simulink model "DPWMA_17_Level_Rectifier_Digital_PR"  (R2023b)
settings: Solver=VariableStepAuto  StartTime=0.0  StopTime=0.5  RelTol=1e-3
libraries: spsDiodeLib x144, spsSeriesRLCBranchLib x39, spsVoltageMeasurementLib x27, spsIGBTDiodeLib x24, simulink x12, spsACVoltageSourceLib x3, spsCurrentMeasurementLib x2, spsMeanLib x2, spsRMSLib x2, slpidlib x1, spsTHDLib x1, spspowerguiLib x1
(part 2 of 2)

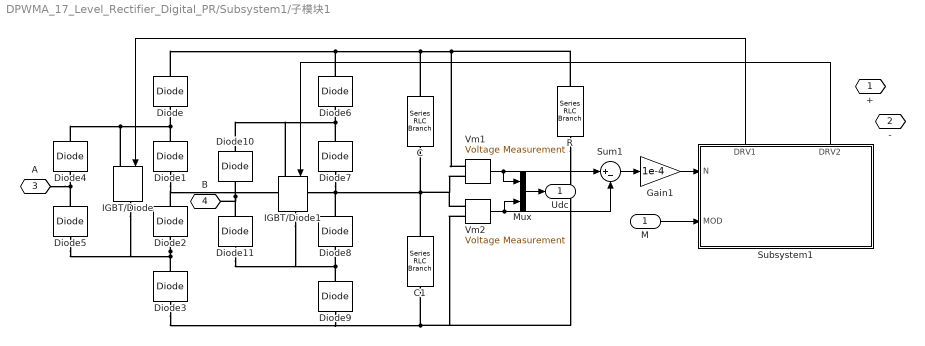
== system DPWMA_17_Level_Rectifier_Digital_PR/Subsystem1/子模块1 ==
  M : Inport
  C : spsSeriesRLCBranchLib/Series RLC Branch  LConnTagsString=__new0  RConnTagsString=__new0  BranchType=C  Resistance=0  Inductance=0  SetiL0=off  InitialCurrent=0  Capacitance=4e-3  Setx0=on  InitialVoltage=860  Measurements=None
  C1 : spsSeriesRLCBranchLib/Series RLC Branch  LConnTagsString=__new0  RConnTagsString=__new0  BranchType=C  Resistance=0  Inductance=0  SetiL0=off  InitialCurrent=0  Capacitance=4e-3  Setx0=on  InitialVoltage=860  Measurements=None
  Diode{,1..3,6..9} (8 alike) : spsDiodeLib/Diode  Ron=0.001  Lon=0  Vf=1.8  IC=0  UseSnubber=0  Rs=5e6  Cs=2e-9  Measurements=off
  Diode{4..5,10..11} (4 alike) : spsDiodeLib/Diode  Ron=0.001  Lon=0  Vf=1  IC=0  UseSnubber=0  Rs=0.05  Cs=1e-8  Measurements=off
  Gain1 : Gain  Gain=1e-4
  IGBT/Diode : spsIGBTDiodeLib/IGBT//Diode  Ron=1e-3  Rs=1e5  Cs=inf  Measurements=off
  IGBT/Diode1 : spsIGBTDiodeLib/IGBT//Diode  Ron=1e-3  Rs=1e5  Cs=inf  Measurements=off
  Mux : Mux  Inputs=2
  R : spsSeriesRLCBranchLib/Series RLC Branch  LConnTagsString=__new0  RConnTagsString=__new0  BranchType=R  Resistance=30  Inductance=0  SetiL0=off  InitialCurrent=0  Capacitance=2e-3  Setx0=on  InitialVoltage=311  Measurements=None
  Subsystem1 : Subsystem
      settings: PortSchema="{\"entries\":[{\"content\":{\"sides\":[{\"content\":{\"connectorIds\":[\"In1\",\"In2\"]},\"type\":\"ConnectorPlacement.EquallySpacedRectSide\",\"uuid\":\"86aef1ad-fbca-44c0-97c4-c9d179baa788\"},{\"content\":{\"side\":\"RIGHT\"},\"type\":\"ConnectorPlacement.EquallySpacedRectSide\",\"uuid\":\"7b15a0f8-39b1-4cc5-afe7-a687626936eb\"},{\"content\":{\"connectorIds\":[\"Out1\",\"Out2\"],\"side\":\"TOP\"},\"type\":\"ConnectorPlacement.EquallySpacedRectSide\",\"uuid\":\"a58ec6d0-3129-4061-af12-e971b5e0e948\"}]},\"type\":\"ConnectorPlacement.EquallySpacedConnector\",\"uuid\":\"d3f7daee-0424-497d-bc41-11931290c6fe\"}],\"packageUris\":[\"http://schema.mathworks.com/mf0/Connector/R2020b\"],\"version\":\"1.0\"}"
  Sum1 : Sum  Inputs=|+-
  Vm1 : spsVoltageMeasurementLib/Voltage Measurement  PhasorSimulation=off  OutputType=Complex  PSBequivalent=0
  Vm2 : spsVoltageMeasurementLib/Voltage Measurement  PhasorSimulation=off  OutputType=Complex  PSBequivalent=0
  + : PMIOPort  Side=Left
  - : PMIOPort  Port=2  Side=Left
  A : PMIOPort  Port=3  Side=Right
  B : PMIOPort  Port=4  Side=Right
  Udc : Outport
  wires:
  Subsystem1/2(DRV2) -> IGBT/Diode1/1
  Subsystem1/1(DRV1) -> IGBT/Diode/1
  M/1 -> Subsystem1/2(MOD)
  Mux/1 -> Udc/1
  Gain1/1 -> Subsystem1/1(N)
  Sum1/1 -> Gain1/1
  Vm2/1 -> Sum1/2, Mux/2
  Vm1/1 -> Sum1/1, Mux/1
  connections:
  Diode10/LConn1 -- B/RConn1 -- Diode11/RConn1
  Diode9/RConn1 -- Diode8/LConn1 -- IGBT/Diode1/RConn1 -- Diode11/LConn1
  Diode7/RConn1 -- Diode6/LConn1 -- Diode10/RConn1 -- IGBT/Diode1/LConn1
  A/RConn1 -- Diode5/RConn1 -- Diode4/LConn1
  Vm2/LConn2 -- R/RConn1 -- Diode3/LConn1 -- Diode9/LConn1 -- C1/RConn1
  Diode2/LConn1 -- Diode3/RConn1 -- Diode5/LConn1 -- IGBT/Diode/RConn1
  Diode4/RConn1 -- IGBT/Diode/LConn1 -- Diode1/RConn1 -- Diode/LConn1
  Diode7/LConn1 -- Diode2/RConn1 -- Diode1/LConn1 -- C/RConn1 -- C1/LConn1 -- Vm2/LConn1 -- Vm1/LConn2 -- Diode8/RConn1
  Diode6/RConn1 -- Diode/RConn1 -- C/LConn1 -- R/LConn1 -- Vm1/LConn1

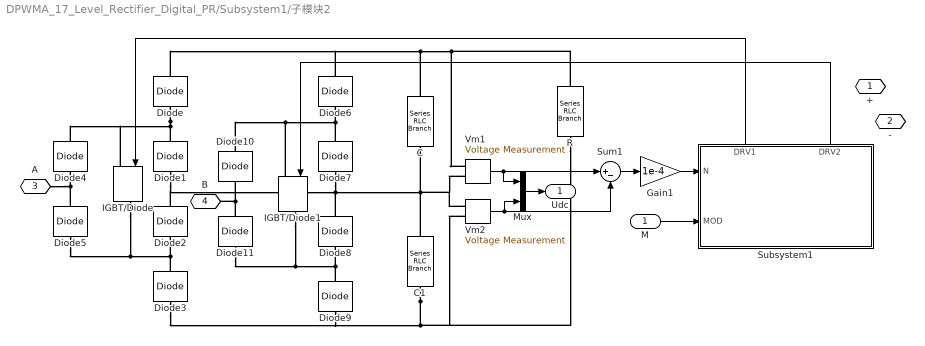
== system DPWMA_17_Level_Rectifier_Digital_PR/Subsystem1/子模块2 ==
  M : Inport
  C : spsSeriesRLCBranchLib/Series RLC Branch  LConnTagsString=__new0  RConnTagsString=__new0  BranchType=C  Resistance=0  Inductance=0  SetiL0=off  InitialCurrent=0  Capacitance=4e-3  Setx0=on  InitialVoltage=850  Measurements=None
  C1 : spsSeriesRLCBranchLib/Series RLC Branch  LConnTagsString=__new0  RConnTagsString=__new0  BranchType=C  Resistance=0  Inductance=0  SetiL0=off  InitialCurrent=0  Capacitance=4e-3  Setx0=on  InitialVoltage=850  Measurements=None
  Diode{,1..3,6..9} (8 alike) : spsDiodeLib/Diode  Ron=0.001  Lon=0  Vf=1.8  IC=0  UseSnubber=0  Rs=5e6  Cs=2e-9  Measurements=off
  Diode{4..5,10..11} (4 alike) : spsDiodeLib/Diode  Ron=0.001  Lon=0  Vf=1  IC=0  UseSnubber=0  Rs=0.05  Cs=1e-8  Measurements=off
  Gain1 : Gain  Gain=1e-4
  IGBT/Diode : spsIGBTDiodeLib/IGBT//Diode  Ron=1e-3  Rs=1e5  Cs=inf  Measurements=off
  IGBT/Diode1 : spsIGBTDiodeLib/IGBT//Diode  Ron=1e-3  Rs=1e5  Cs=inf  Measurements=off
  Mux : Mux  Inputs=2
  R : spsSeriesRLCBranchLib/Series RLC Branch  LConnTagsString=__new0  RConnTagsString=__new0  BranchType=R  Resistance=30  Inductance=0  SetiL0=off  InitialCurrent=0  Capacitance=2e-3  Setx0=on  InitialVoltage=311  Measurements=None
  Subsystem1 : Subsystem
      settings: PortSchema="{\"entries\":[{\"content\":{\"sides\":[{\"content\":{\"connectorIds\":[\"In1\",\"In2\"]},\"type\":\"ConnectorPlacement.EquallySpacedRectSide\",\"uuid\":\"86aef1ad-fbca-44c0-97c4-c9d179baa788\"},{\"content\":{\"side\":\"RIGHT\"},\"type\":\"ConnectorPlacement.EquallySpacedRectSide\",\"uuid\":\"7b15a0f8-39b1-4cc5-afe7-a687626936eb\"},{\"content\":{\"connectorIds\":[\"Out1\",\"Out2\"],\"side\":\"TOP\"},\"type\":\"ConnectorPlacement.EquallySpacedRectSide\",\"uuid\":\"a58ec6d0-3129-4061-af12-e971b5e0e948\"}]},\"type\":\"ConnectorPlacement.EquallySpacedConnector\",\"uuid\":\"d3f7daee-0424-497d-bc41-11931290c6fe\"}],\"packageUris\":[\"http://schema.mathworks.com/mf0/Connector/R2020b\"],\"version\":\"1.0\"}"
  Sum1 : Sum  Inputs=|+-
  Vm1 : spsVoltageMeasurementLib/Voltage Measurement  PhasorSimulation=off  OutputType=Complex  PSBequivalent=0
  Vm2 : spsVoltageMeasurementLib/Voltage Measurement  PhasorSimulation=off  OutputType=Complex  PSBequivalent=0
  + : PMIOPort  Side=Left
  - : PMIOPort  Port=2  Side=Left
  A : PMIOPort  Port=3  Side=Right
  B : PMIOPort  Port=4  Side=Right
  Udc : Outport
  wires:
  Vm1/1 -> Mux/1, Sum1/1
  Vm2/1 -> Mux/2, Sum1/2
  Sum1/1 -> Gain1/1
  Gain1/1 -> Subsystem1/1(N)
  Mux/1 -> Udc/1
  M/1 -> Subsystem1/2(MOD)
  Subsystem1/1(DRV1) -> IGBT/Diode/1
  Subsystem1/2(DRV2) -> IGBT/Diode1/1
  connections:
  Vm1/LConn1 -- R/LConn1 -- C/LConn1 -- Diode/RConn1 -- Diode6/RConn1
  Diode8/RConn1 -- Vm1/LConn2 -- Vm2/LConn1 -- C1/LConn1 -- C/RConn1 -- Diode1/LConn1 -- Diode2/RConn1 -- Diode7/LConn1
  Diode/LConn1 -- Diode1/RConn1 -- IGBT/Diode/LConn1 -- Diode4/RConn1
  IGBT/Diode/RConn1 -- Diode5/LConn1 -- Diode3/RConn1 -- Diode2/LConn1
  C1/RConn1 -- Diode9/LConn1 -- Diode3/LConn1 -- R/RConn1 -- Vm2/LConn2
  Diode4/LConn1 -- Diode5/RConn1 -- A/RConn1
  IGBT/Diode1/LConn1 -- Diode10/RConn1 -- Diode6/LConn1 -- Diode7/RConn1
  Diode11/LConn1 -- IGBT/Diode1/RConn1 -- Diode8/LConn1 -- Diode9/RConn1
  Diode11/RConn1 -- B/RConn1 -- Diode10/LConn1

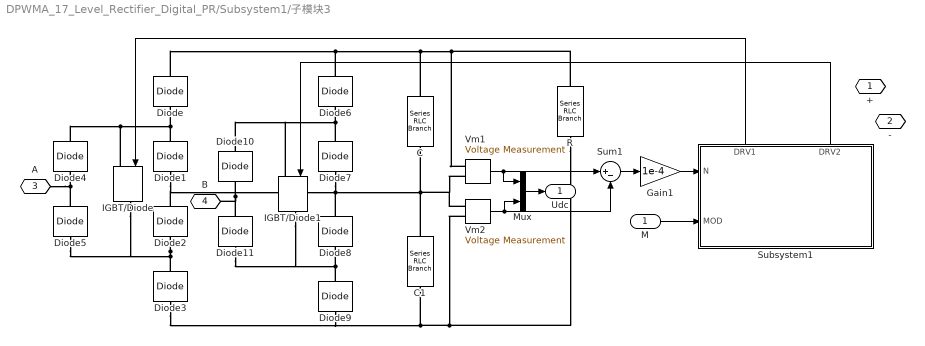
== system DPWMA_17_Level_Rectifier_Digital_PR/Subsystem1/子模块3 ==
  M : Inport
  C : spsSeriesRLCBranchLib/Series RLC Branch  LConnTagsString=__new0  RConnTagsString=__new0  BranchType=C  Resistance=0  Inductance=0  SetiL0=off  InitialCurrent=0  Capacitance=4e-3  Setx0=on  InitialVoltage=850  Measurements=None
  C1 : spsSeriesRLCBranchLib/Series RLC Branch  LConnTagsString=__new0  RConnTagsString=__new0  BranchType=C  Resistance=0  Inductance=0  SetiL0=off  InitialCurrent=0  Capacitance=4e-3  Setx0=on  InitialVoltage=850  Measurements=None
  Diode{,1..3,6..9} (8 alike) : spsDiodeLib/Diode  Ron=0.001  Lon=0  Vf=1.8  IC=0  UseSnubber=0  Rs=5e6  Cs=2e-9  Measurements=off
  Diode{4..5,10..11} (4 alike) : spsDiodeLib/Diode  Ron=0.001  Lon=0  Vf=1  IC=0  UseSnubber=0  Rs=0.05  Cs=1e-8  Measurements=off
  Gain1 : Gain  Gain=1e-4
  IGBT/Diode : spsIGBTDiodeLib/IGBT//Diode  Ron=1e-3  Rs=1e5  Cs=inf  Measurements=off
  IGBT/Diode1 : spsIGBTDiodeLib/IGBT//Diode  Ron=1e-3  Rs=1e5  Cs=inf  Measurements=off
  Mux : Mux  Inputs=2
  R : spsSeriesRLCBranchLib/Series RLC Branch  LConnTagsString=__new0  RConnTagsString=__new0  BranchType=R  Resistance=30  Inductance=0  SetiL0=off  InitialCurrent=0  Capacitance=2e-3  Setx0=on  InitialVoltage=311  Measurements=None
  Subsystem1 : Subsystem
      settings: PortSchema="{\"entries\":[{\"content\":{\"sides\":[{\"content\":{\"connectorIds\":[\"In1\",\"In2\"]},\"type\":\"ConnectorPlacement.EquallySpacedRectSide\",\"uuid\":\"86aef1ad-fbca-44c0-97c4-c9d179baa788\"},{\"content\":{\"side\":\"RIGHT\"},\"type\":\"ConnectorPlacement.EquallySpacedRectSide\",\"uuid\":\"7b15a0f8-39b1-4cc5-afe7-a687626936eb\"},{\"content\":{\"connectorIds\":[\"Out1\",\"Out2\"],\"side\":\"TOP\"},\"type\":\"ConnectorPlacement.EquallySpacedRectSide\",\"uuid\":\"a58ec6d0-3129-4061-af12-e971b5e0e948\"}]},\"type\":\"ConnectorPlacement.EquallySpacedConnector\",\"uuid\":\"d3f7daee-0424-497d-bc41-11931290c6fe\"}],\"packageUris\":[\"http://schema.mathworks.com/mf0/Connector/R2020b\"],\"version\":\"1.0\"}"
  Sum1 : Sum  Inputs=|+-
  Vm1 : spsVoltageMeasurementLib/Voltage Measurement  PhasorSimulation=off  OutputType=Complex  PSBequivalent=0
  Vm2 : spsVoltageMeasurementLib/Voltage Measurement  PhasorSimulation=off  OutputType=Complex  PSBequivalent=0
  + : PMIOPort  Side=Left
  - : PMIOPort  Port=2  Side=Left
  A : PMIOPort  Port=3  Side=Right
  B : PMIOPort  Port=4  Side=Right
  Udc : Outport
  wires:
  Subsystem1/2(DRV2) -> IGBT/Diode1/1
  Subsystem1/1(DRV1) -> IGBT/Diode/1
  M/1 -> Subsystem1/2(MOD)
  Mux/1 -> Udc/1
  Gain1/1 -> Subsystem1/1(N)
  Sum1/1 -> Gain1/1
  Vm2/1 -> Sum1/2, Mux/2
  Vm1/1 -> Sum1/1, Mux/1
  connections:
  Diode10/LConn1 -- B/RConn1 -- Diode11/RConn1
  Diode9/RConn1 -- Diode8/LConn1 -- IGBT/Diode1/RConn1 -- Diode11/LConn1
  Diode7/RConn1 -- Diode6/LConn1 -- Diode10/RConn1 -- IGBT/Diode1/LConn1
  A/RConn1 -- Diode5/RConn1 -- Diode4/LConn1
  Vm2/LConn2 -- R/RConn1 -- Diode3/LConn1 -- Diode9/LConn1 -- C1/RConn1
  Diode2/LConn1 -- Diode3/RConn1 -- Diode5/LConn1 -- IGBT/Diode/RConn1
  Diode4/RConn1 -- IGBT/Diode/LConn1 -- Diode1/RConn1 -- Diode/LConn1
  Diode7/LConn1 -- Diode2/RConn1 -- Diode1/LConn1 -- C/RConn1 -- C1/LConn1 -- Vm2/LConn1 -- Vm1/LConn2 -- Diode8/RConn1
  Diode6/RConn1 -- Diode/RConn1 -- C/LConn1 -- R/LConn1 -- Vm1/LConn1

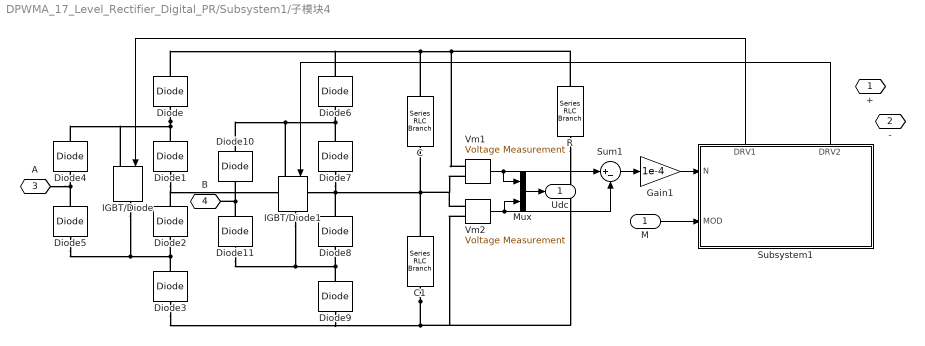
== system DPWMA_17_Level_Rectifier_Digital_PR/Subsystem1/子模块4 ==
  M : Inport
  C : spsSeriesRLCBranchLib/Series RLC Branch  LConnTagsString=__new0  RConnTagsString=__new0  BranchType=C  Resistance=0  Inductance=0  SetiL0=off  InitialCurrent=0  Capacitance=4e-3  Setx0=on  InitialVoltage=850  Measurements=None
  C1 : spsSeriesRLCBranchLib/Series RLC Branch  LConnTagsString=__new0  RConnTagsString=__new0  BranchType=C  Resistance=0  Inductance=0  SetiL0=off  InitialCurrent=0  Capacitance=4e-3  Setx0=on  InitialVoltage=850  Measurements=None
  Diode{,1..3,6..9} (8 alike) : spsDiodeLib/Diode  Ron=0.001  Lon=0  Vf=1.8  IC=0  UseSnubber=0  Rs=5e6  Cs=2e-9  Measurements=off
  Diode{4..5,10..11} (4 alike) : spsDiodeLib/Diode  Ron=0.001  Lon=0  Vf=1  IC=0  UseSnubber=0  Rs=0.05  Cs=1e-8  Measurements=off
  Gain1 : Gain  Gain=1e-4
  IGBT/Diode : spsIGBTDiodeLib/IGBT//Diode  Ron=1e-3  Rs=1e5  Cs=inf  Measurements=off
  IGBT/Diode1 : spsIGBTDiodeLib/IGBT//Diode  Ron=1e-3  Rs=1e5  Cs=inf  Measurements=off
  Mux : Mux  Inputs=2
  R : spsSeriesRLCBranchLib/Series RLC Branch  LConnTagsString=__new0  RConnTagsString=__new0  BranchType=R  Resistance=30  Inductance=0  SetiL0=off  InitialCurrent=0  Capacitance=2e-3  Setx0=on  InitialVoltage=311  Measurements=None
  Subsystem1 : Subsystem
      settings: PortSchema="{\"entries\":[{\"content\":{\"sides\":[{\"content\":{\"connectorIds\":[\"In1\",\"In2\"]},\"type\":\"ConnectorPlacement.EquallySpacedRectSide\",\"uuid\":\"86aef1ad-fbca-44c0-97c4-c9d179baa788\"},{\"content\":{\"side\":\"RIGHT\"},\"type\":\"ConnectorPlacement.EquallySpacedRectSide\",\"uuid\":\"7b15a0f8-39b1-4cc5-afe7-a687626936eb\"},{\"content\":{\"connectorIds\":[\"Out1\",\"Out2\"],\"side\":\"TOP\"},\"type\":\"ConnectorPlacement.EquallySpacedRectSide\",\"uuid\":\"a58ec6d0-3129-4061-af12-e971b5e0e948\"}]},\"type\":\"ConnectorPlacement.EquallySpacedConnector\",\"uuid\":\"d3f7daee-0424-497d-bc41-11931290c6fe\"}],\"packageUris\":[\"http://schema.mathworks.com/mf0/Connector/R2020b\"],\"version\":\"1.0\"}"
  Sum1 : Sum  Inputs=|+-
  Vm1 : spsVoltageMeasurementLib/Voltage Measurement  PhasorSimulation=off  OutputType=Complex  PSBequivalent=0
  Vm2 : spsVoltageMeasurementLib/Voltage Measurement  PhasorSimulation=off  OutputType=Complex  PSBequivalent=0
  + : PMIOPort  Side=Left
  - : PMIOPort  Port=2  Side=Left
  A : PMIOPort  Port=3  Side=Right
  B : PMIOPort  Port=4  Side=Right
  Udc : Outport
  wires:
  Vm1/1 -> Mux/1, Sum1/1
  Vm2/1 -> Mux/2, Sum1/2
  Sum1/1 -> Gain1/1
  Gain1/1 -> Subsystem1/1(N)
  Mux/1 -> Udc/1
  M/1 -> Subsystem1/2(MOD)
  Subsystem1/1(DRV1) -> IGBT/Diode/1
  Subsystem1/2(DRV2) -> IGBT/Diode1/1
  connections:
  Vm1/LConn1 -- R/LConn1 -- C/LConn1 -- Diode/RConn1 -- Diode6/RConn1
  Diode8/RConn1 -- Vm1/LConn2 -- Vm2/LConn1 -- C1/LConn1 -- C/RConn1 -- Diode1/LConn1 -- Diode2/RConn1 -- Diode7/LConn1
  Diode/LConn1 -- Diode1/RConn1 -- IGBT/Diode/LConn1 -- Diode4/RConn1
  IGBT/Diode/RConn1 -- Diode5/LConn1 -- Diode3/RConn1 -- Diode2/LConn1
  C1/RConn1 -- Diode9/LConn1 -- Diode3/LConn1 -- R/RConn1 -- Vm2/LConn2
  Diode4/LConn1 -- Diode5/RConn1 -- A/RConn1
  IGBT/Diode1/LConn1 -- Diode10/RConn1 -- Diode6/LConn1 -- Diode7/RConn1
  Diode11/LConn1 -- IGBT/Diode1/RConn1 -- Diode8/LConn1 -- Diode9/RConn1
  Diode11/RConn1 -- B/RConn1 -- Diode10/LConn1

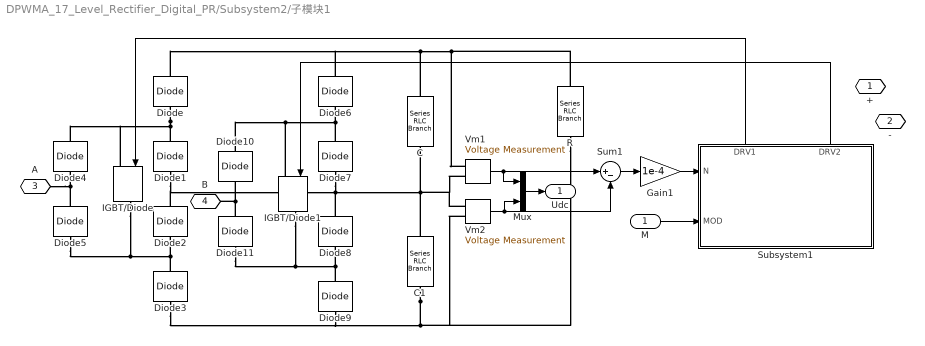
== system DPWMA_17_Level_Rectifier_Digital_PR/Subsystem2/子模块1 ==
  M : Inport
  C : spsSeriesRLCBranchLib/Series RLC Branch  LConnTagsString=__new0  RConnTagsString=__new0  BranchType=C  Resistance=0  Inductance=0  SetiL0=off  InitialCurrent=0  Capacitance=4e-3  Setx0=on  InitialVoltage=860  Measurements=None
  C1 : spsSeriesRLCBranchLib/Series RLC Branch  LConnTagsString=__new0  RConnTagsString=__new0  BranchType=C  Resistance=0  Inductance=0  SetiL0=off  InitialCurrent=0  Capacitance=4e-3  Setx0=on  InitialVoltage=860  Measurements=None
  Diode{,1..3,6..9} (8 alike) : spsDiodeLib/Diode  Ron=0.001  Lon=0  Vf=1.8  IC=0  UseSnubber=0  Rs=5e6  Cs=2e-9  Measurements=off
  Diode{4..5,10..11} (4 alike) : spsDiodeLib/Diode  Ron=0.001  Lon=0  Vf=1  IC=0  UseSnubber=0  Rs=0.05  Cs=1e-8  Measurements=off
  Gain1 : Gain  Gain=1e-4
  IGBT/Diode : spsIGBTDiodeLib/IGBT//Diode  Ron=1e-3  Rs=1e5  Cs=inf  Measurements=off
  IGBT/Diode1 : spsIGBTDiodeLib/IGBT//Diode  Ron=1e-3  Rs=1e5  Cs=inf  Measurements=off
  Mux : Mux  Inputs=2
  R : spsSeriesRLCBranchLib/Series RLC Branch  LConnTagsString=__new0  RConnTagsString=__new0  BranchType=R  Resistance=30  Inductance=0  SetiL0=off  InitialCurrent=0  Capacitance=2e-3  Setx0=on  InitialVoltage=311  Measurements=None
  Subsystem1 : Subsystem
      settings: PortSchema="{\"entries\":[{\"content\":{\"sides\":[{\"content\":{\"connectorIds\":[\"In1\",\"In2\"]},\"type\":\"ConnectorPlacement.EquallySpacedRectSide\",\"uuid\":\"86aef1ad-fbca-44c0-97c4-c9d179baa788\"},{\"content\":{\"side\":\"RIGHT\"},\"type\":\"ConnectorPlacement.EquallySpacedRectSide\",\"uuid\":\"7b15a0f8-39b1-4cc5-afe7-a687626936eb\"},{\"content\":{\"connectorIds\":[\"Out1\",\"Out2\"],\"side\":\"TOP\"},\"type\":\"ConnectorPlacement.EquallySpacedRectSide\",\"uuid\":\"a58ec6d0-3129-4061-af12-e971b5e0e948\"}]},\"type\":\"ConnectorPlacement.EquallySpacedConnector\",\"uuid\":\"d3f7daee-0424-497d-bc41-11931290c6fe\"}],\"packageUris\":[\"http://schema.mathworks.com/mf0/Connector/R2020b\"],\"version\":\"1.0\"}"
  Sum1 : Sum  Inputs=|+-
  Vm1 : spsVoltageMeasurementLib/Voltage Measurement  PhasorSimulation=off  OutputType=Complex  PSBequivalent=0
  Vm2 : spsVoltageMeasurementLib/Voltage Measurement  PhasorSimulation=off  OutputType=Complex  PSBequivalent=0
  + : PMIOPort  Side=Left
  - : PMIOPort  Port=2  Side=Left
  A : PMIOPort  Port=3  Side=Right
  B : PMIOPort  Port=4  Side=Right
  Udc : Outport
  wires:
  Vm1/1 -> Mux/1, Sum1/1
  Vm2/1 -> Mux/2, Sum1/2
  Sum1/1 -> Gain1/1
  Gain1/1 -> Subsystem1/1(N)
  Mux/1 -> Udc/1
  M/1 -> Subsystem1/2(MOD)
  Subsystem1/1(DRV1) -> IGBT/Diode/1
  Subsystem1/2(DRV2) -> IGBT/Diode1/1
  connections:
  Vm1/LConn1 -- R/LConn1 -- C/LConn1 -- Diode/RConn1 -- Diode6/RConn1
  Diode8/RConn1 -- Vm1/LConn2 -- Vm2/LConn1 -- C1/LConn1 -- C/RConn1 -- Diode1/LConn1 -- Diode2/RConn1 -- Diode7/LConn1
  Diode/LConn1 -- Diode1/RConn1 -- IGBT/Diode/LConn1 -- Diode4/RConn1
  IGBT/Diode/RConn1 -- Diode5/LConn1 -- Diode3/RConn1 -- Diode2/LConn1
  C1/RConn1 -- Diode9/LConn1 -- Diode3/LConn1 -- R/RConn1 -- Vm2/LConn2
  Diode4/LConn1 -- Diode5/RConn1 -- A/RConn1
  IGBT/Diode1/LConn1 -- Diode10/RConn1 -- Diode6/LConn1 -- Diode7/RConn1
  Diode11/LConn1 -- IGBT/Diode1/RConn1 -- Diode8/LConn1 -- Diode9/RConn1
  Diode11/RConn1 -- B/RConn1 -- Diode10/LConn1

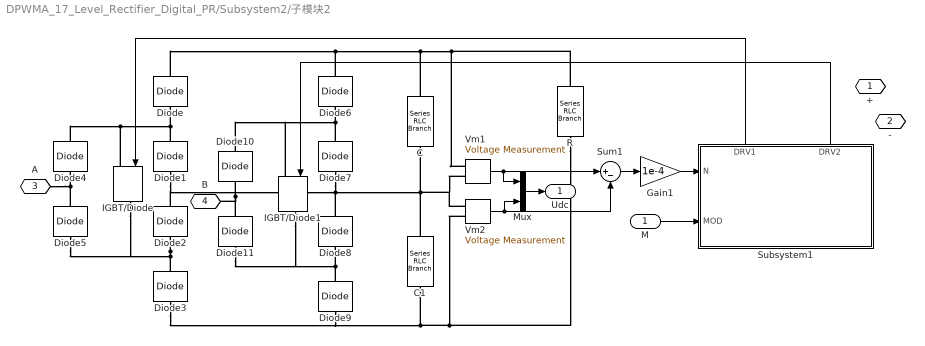
== system DPWMA_17_Level_Rectifier_Digital_PR/Subsystem2/子模块2 ==
  M : Inport
  C : spsSeriesRLCBranchLib/Series RLC Branch  LConnTagsString=__new0  RConnTagsString=__new0  BranchType=C  Resistance=0  Inductance=0  SetiL0=off  InitialCurrent=0  Capacitance=4e-3  Setx0=on  InitialVoltage=850  Measurements=None
  C1 : spsSeriesRLCBranchLib/Series RLC Branch  LConnTagsString=__new0  RConnTagsString=__new0  BranchType=C  Resistance=0  Inductance=0  SetiL0=off  InitialCurrent=0  Capacitance=4e-3  Setx0=on  InitialVoltage=850  Measurements=None
  Diode{,1..3,6..9} (8 alike) : spsDiodeLib/Diode  Ron=0.001  Lon=0  Vf=1.8  IC=0  UseSnubber=0  Rs=5e6  Cs=2e-9  Measurements=off
  Diode{4..5,10..11} (4 alike) : spsDiodeLib/Diode  Ron=0.001  Lon=0  Vf=1  IC=0  UseSnubber=0  Rs=0.05  Cs=1e-8  Measurements=off
  Gain1 : Gain  Gain=1e-4
  IGBT/Diode : spsIGBTDiodeLib/IGBT//Diode  Ron=1e-3  Rs=1e5  Cs=inf  Measurements=off
  IGBT/Diode1 : spsIGBTDiodeLib/IGBT//Diode  Ron=1e-3  Rs=1e5  Cs=inf  Measurements=off
  Mux : Mux  Inputs=2
  R : spsSeriesRLCBranchLib/Series RLC Branch  LConnTagsString=__new0  RConnTagsString=__new0  BranchType=R  Resistance=30  Inductance=0  SetiL0=off  InitialCurrent=0  Capacitance=2e-3  Setx0=on  InitialVoltage=311  Measurements=None
  Subsystem1 : Subsystem
      settings: PortSchema="{\"entries\":[{\"content\":{\"sides\":[{\"content\":{\"connectorIds\":[\"In1\",\"In2\"]},\"type\":\"ConnectorPlacement.EquallySpacedRectSide\",\"uuid\":\"86aef1ad-fbca-44c0-97c4-c9d179baa788\"},{\"content\":{\"side\":\"RIGHT\"},\"type\":\"ConnectorPlacement.EquallySpacedRectSide\",\"uuid\":\"7b15a0f8-39b1-4cc5-afe7-a687626936eb\"},{\"content\":{\"connectorIds\":[\"Out1\",\"Out2\"],\"side\":\"TOP\"},\"type\":\"ConnectorPlacement.EquallySpacedRectSide\",\"uuid\":\"a58ec6d0-3129-4061-af12-e971b5e0e948\"}]},\"type\":\"ConnectorPlacement.EquallySpacedConnector\",\"uuid\":\"d3f7daee-0424-497d-bc41-11931290c6fe\"}],\"packageUris\":[\"http://schema.mathworks.com/mf0/Connector/R2020b\"],\"version\":\"1.0\"}"
  Sum1 : Sum  Inputs=|+-
  Vm1 : spsVoltageMeasurementLib/Voltage Measurement  PhasorSimulation=off  OutputType=Complex  PSBequivalent=0
  Vm2 : spsVoltageMeasurementLib/Voltage Measurement  PhasorSimulation=off  OutputType=Complex  PSBequivalent=0
  + : PMIOPort  Side=Left
  - : PMIOPort  Port=2  Side=Left
  A : PMIOPort  Port=3  Side=Right
  B : PMIOPort  Port=4  Side=Right
  Udc : Outport
  wires:
  Subsystem1/2(DRV2) -> IGBT/Diode1/1
  Subsystem1/1(DRV1) -> IGBT/Diode/1
  M/1 -> Subsystem1/2(MOD)
  Mux/1 -> Udc/1
  Gain1/1 -> Subsystem1/1(N)
  Sum1/1 -> Gain1/1
  Vm2/1 -> Sum1/2, Mux/2
  Vm1/1 -> Sum1/1, Mux/1
  connections:
  Diode10/LConn1 -- B/RConn1 -- Diode11/RConn1
  Diode9/RConn1 -- Diode8/LConn1 -- IGBT/Diode1/RConn1 -- Diode11/LConn1
  Diode7/RConn1 -- Diode6/LConn1 -- Diode10/RConn1 -- IGBT/Diode1/LConn1
  A/RConn1 -- Diode5/RConn1 -- Diode4/LConn1
  Vm2/LConn2 -- R/RConn1 -- Diode3/LConn1 -- Diode9/LConn1 -- C1/RConn1
  Diode2/LConn1 -- Diode3/RConn1 -- Diode5/LConn1 -- IGBT/Diode/RConn1
  Diode4/RConn1 -- IGBT/Diode/LConn1 -- Diode1/RConn1 -- Diode/LConn1
  Diode7/LConn1 -- Diode2/RConn1 -- Diode1/LConn1 -- C/RConn1 -- C1/LConn1 -- Vm2/LConn1 -- Vm1/LConn2 -- Diode8/RConn1
  Diode6/RConn1 -- Diode/RConn1 -- C/LConn1 -- R/LConn1 -- Vm1/LConn1

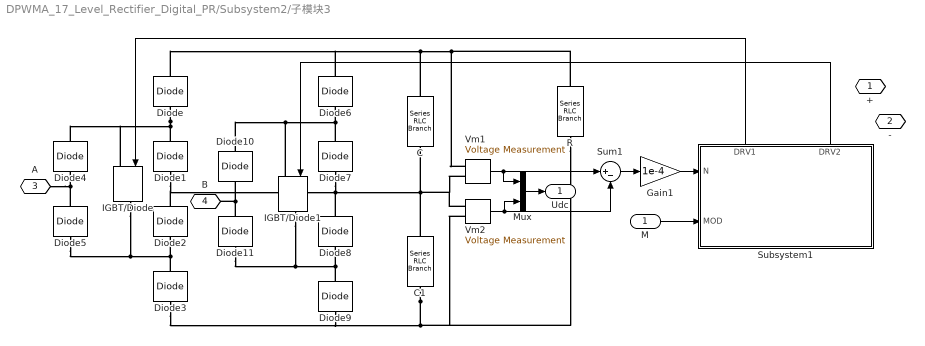
== system DPWMA_17_Level_Rectifier_Digital_PR/Subsystem2/子模块3 ==
  M : Inport
  C : spsSeriesRLCBranchLib/Series RLC Branch  LConnTagsString=__new0  RConnTagsString=__new0  BranchType=C  Resistance=0  Inductance=0  SetiL0=off  InitialCurrent=0  Capacitance=4e-3  Setx0=on  InitialVoltage=850  Measurements=None
  C1 : spsSeriesRLCBranchLib/Series RLC Branch  LConnTagsString=__new0  RConnTagsString=__new0  BranchType=C  Resistance=0  Inductance=0  SetiL0=off  InitialCurrent=0  Capacitance=4e-3  Setx0=on  InitialVoltage=850  Measurements=None
  Diode{,1..3,6..9} (8 alike) : spsDiodeLib/Diode  Ron=0.001  Lon=0  Vf=1.8  IC=0  UseSnubber=0  Rs=5e6  Cs=2e-9  Measurements=off
  Diode{4..5,10..11} (4 alike) : spsDiodeLib/Diode  Ron=0.001  Lon=0  Vf=1  IC=0  UseSnubber=0  Rs=0.05  Cs=1e-8  Measurements=off
  Gain1 : Gain  Gain=1e-4
  IGBT/Diode : spsIGBTDiodeLib/IGBT//Diode  Ron=1e-3  Rs=1e5  Cs=inf  Measurements=off
  IGBT/Diode1 : spsIGBTDiodeLib/IGBT//Diode  Ron=1e-3  Rs=1e5  Cs=inf  Measurements=off
  Mux : Mux  Inputs=2
  R : spsSeriesRLCBranchLib/Series RLC Branch  LConnTagsString=__new0  RConnTagsString=__new0  BranchType=R  Resistance=30  Inductance=0  SetiL0=off  InitialCurrent=0  Capacitance=2e-3  Setx0=on  InitialVoltage=311  Measurements=None
  Subsystem1 : Subsystem
      settings: PortSchema="{\"entries\":[{\"content\":{\"sides\":[{\"content\":{\"connectorIds\":[\"In1\",\"In2\"]},\"type\":\"ConnectorPlacement.EquallySpacedRectSide\",\"uuid\":\"86aef1ad-fbca-44c0-97c4-c9d179baa788\"},{\"content\":{\"side\":\"RIGHT\"},\"type\":\"ConnectorPlacement.EquallySpacedRectSide\",\"uuid\":\"7b15a0f8-39b1-4cc5-afe7-a687626936eb\"},{\"content\":{\"connectorIds\":[\"Out1\",\"Out2\"],\"side\":\"TOP\"},\"type\":\"ConnectorPlacement.EquallySpacedRectSide\",\"uuid\":\"a58ec6d0-3129-4061-af12-e971b5e0e948\"}]},\"type\":\"ConnectorPlacement.EquallySpacedConnector\",\"uuid\":\"d3f7daee-0424-497d-bc41-11931290c6fe\"}],\"packageUris\":[\"http://schema.mathworks.com/mf0/Connector/R2020b\"],\"version\":\"1.0\"}"
  Sum1 : Sum  Inputs=|+-
  Vm1 : spsVoltageMeasurementLib/Voltage Measurement  PhasorSimulation=off  OutputType=Complex  PSBequivalent=0
  Vm2 : spsVoltageMeasurementLib/Voltage Measurement  PhasorSimulation=off  OutputType=Complex  PSBequivalent=0
  + : PMIOPort  Side=Left
  - : PMIOPort  Port=2  Side=Left
  A : PMIOPort  Port=3  Side=Right
  B : PMIOPort  Port=4  Side=Right
  Udc : Outport
  wires:
  Vm1/1 -> Mux/1, Sum1/1
  Vm2/1 -> Mux/2, Sum1/2
  Sum1/1 -> Gain1/1
  Gain1/1 -> Subsystem1/1(N)
  Mux/1 -> Udc/1
  M/1 -> Subsystem1/2(MOD)
  Subsystem1/1(DRV1) -> IGBT/Diode/1
  Subsystem1/2(DRV2) -> IGBT/Diode1/1
  connections:
  Vm1/LConn1 -- R/LConn1 -- C/LConn1 -- Diode/RConn1 -- Diode6/RConn1
  Diode8/RConn1 -- Vm1/LConn2 -- Vm2/LConn1 -- C1/LConn1 -- C/RConn1 -- Diode1/LConn1 -- Diode2/RConn1 -- Diode7/LConn1
  Diode/LConn1 -- Diode1/RConn1 -- IGBT/Diode/LConn1 -- Diode4/RConn1
  IGBT/Diode/RConn1 -- Diode5/LConn1 -- Diode3/RConn1 -- Diode2/LConn1
  C1/RConn1 -- Diode9/LConn1 -- Diode3/LConn1 -- R/RConn1 -- Vm2/LConn2
  Diode4/LConn1 -- Diode5/RConn1 -- A/RConn1
  IGBT/Diode1/LConn1 -- Diode10/RConn1 -- Diode6/LConn1 -- Diode7/RConn1
  Diode11/LConn1 -- IGBT/Diode1/RConn1 -- Diode8/LConn1 -- Diode9/RConn1
  Diode11/RConn1 -- B/RConn1 -- Diode10/LConn1

== system DPWMA_17_Level_Rectifier_Digital_PR/Subsystem2/子模块4 ==
  M : Inport
  C : spsSeriesRLCBranchLib/Series RLC Branch  LConnTagsString=__new0  RConnTagsString=__new0  BranchType=C  Resistance=0  Inductance=0  SetiL0=off  InitialCurrent=0  Capacitance=4e-3  Setx0=on  InitialVoltage=850  Measurements=None
  C1 : spsSeriesRLCBranchLib/Series RLC Branch  LConnTagsString=__new0  RConnTagsString=__new0  BranchType=C  Resistance=0  Inductance=0  SetiL0=off  InitialCurrent=0  Capacitance=4e-3  Setx0=on  InitialVoltage=850  Measurements=None
  Diode{,1..3,6..9} (8 alike) : spsDiodeLib/Diode  Ron=0.001  Lon=0  Vf=1.8  IC=0  UseSnubber=0  Rs=5e6  Cs=2e-9  Measurements=off
  Diode{4..5,10..11} (4 alike) : spsDiodeLib/Diode  Ron=0.001  Lon=0  Vf=1  IC=0  UseSnubber=0  Rs=0.05  Cs=1e-8  Measurements=off
  Gain1 : Gain  Gain=1e-4
  IGBT/Diode : spsIGBTDiodeLib/IGBT//Diode  Ron=1e-3  Rs=1e5  Cs=inf  Measurements=off
  IGBT/Diode1 : spsIGBTDiodeLib/IGBT//Diode  Ron=1e-3  Rs=1e5  Cs=inf  Measurements=off
  Mux : Mux  Inputs=2
  R : spsSeriesRLCBranchLib/Series RLC Branch  LConnTagsString=__new0  RConnTagsString=__new0  BranchType=R  Resistance=30  Inductance=0  SetiL0=off  InitialCurrent=0  Capacitance=2e-3  Setx0=on  InitialVoltage=311  Measurements=None
  Subsystem1 : Subsystem
      settings: PortSchema="{\"entries\":[{\"content\":{\"sides\":[{\"content\":{\"connectorIds\":[\"In1\",\"In2\"]},\"type\":\"ConnectorPlacement.EquallySpacedRectSide\",\"uuid\":\"86aef1ad-fbca-44c0-97c4-c9d179baa788\"},{\"content\":{\"side\":\"RIGHT\"},\"type\":\"ConnectorPlacement.EquallySpacedRectSide\",\"uuid\":\"7b15a0f8-39b1-4cc5-afe7-a687626936eb\"},{\"content\":{\"connectorIds\":[\"Out1\",\"Out2\"],\"side\":\"TOP\"},\"type\":\"ConnectorPlacement.EquallySpacedRectSide\",\"uuid\":\"a58ec6d0-3129-4061-af12-e971b5e0e948\"}]},\"type\":\"ConnectorPlacement.EquallySpacedConnector\",\"uuid\":\"d3f7daee-0424-497d-bc41-11931290c6fe\"}],\"packageUris\":[\"http://schema.mathworks.com/mf0/Connector/R2020b\"],\"version\":\"1.0\"}"
  Sum1 : Sum  Inputs=|+-
  Vm1 : spsVoltageMeasurementLib/Voltage Measurement  PhasorSimulation=off  OutputType=Complex  PSBequivalent=0
  Vm2 : spsVoltageMeasurementLib/Voltage Measurement  PhasorSimulation=off  OutputType=Complex  PSBequivalent=0
  + : PMIOPort  Side=Left
  - : PMIOPort  Port=2  Side=Left
  A : PMIOPort  Port=3  Side=Right
  B : PMIOPort  Port=4  Side=Right
  Udc : Outport
  wires:
  Subsystem1/2(DRV2) -> IGBT/Diode1/1
  Subsystem1/1(DRV1) -> IGBT/Diode/1
  M/1 -> Subsystem1/2(MOD)
  Mux/1 -> Udc/1
  Gain1/1 -> Subsystem1/1(N)
  Sum1/1 -> Gain1/1
  Vm2/1 -> Sum1/2, Mux/2
  Vm1/1 -> Sum1/1, Mux/1
  connections:
  Diode10/LConn1 -- B/RConn1 -- Diode11/RConn1
  Diode9/RConn1 -- Diode8/LConn1 -- IGBT/Diode1/RConn1 -- Diode11/LConn1
  Diode7/RConn1 -- Diode6/LConn1 -- Diode10/RConn1 -- IGBT/Diode1/LConn1
  A/RConn1 -- Diode5/RConn1 -- Diode4/LConn1
  Vm2/LConn2 -- R/RConn1 -- Diode3/LConn1 -- Diode9/LConn1 -- C1/RConn1
  Diode2/LConn1 -- Diode3/RConn1 -- Diode5/LConn1 -- IGBT/Diode/RConn1
  Diode4/RConn1 -- IGBT/Diode/LConn1 -- Diode1/RConn1 -- Diode/LConn1
  Diode7/LConn1 -- Diode2/RConn1 -- Diode1/LConn1 -- C/RConn1 -- C1/LConn1 -- Vm2/LConn1 -- Vm1/LConn2 -- Diode8/RConn1
  Diode6/RConn1 -- Diode/RConn1 -- C/LConn1 -- R/LConn1 -- Vm1/LConn1

== system DPWMA_17_Level_Rectifier_Digital_PR/Subsystem3/QuTrans ==
  ac : Inport
  Demux : Demux  Outputs=2
  Mux : Mux  Inputs=3
  Sum6 : Sum  Inputs=-|-
  abc : Outport
  wires:
  ac/1 -> Demux/1
  Sum6/1 -> Mux/2
  Demux/1 -> Sum6/1, Mux/1
  Demux/2 -> Sum6/2, Mux/3
  Mux/1 -> abc/1

== system DPWMA_17_Level_Rectifier_Digital_PR/Subsystem3/QuTrans1 ==
  ac : Inport
  Demux : Demux  Outputs=2
  Mux : Mux  Inputs=3
  Sum6 : Sum  Inputs=-|-
  abc : Outport
  wires:
  Mux/1 -> abc/1
  Demux/2 -> Mux/3, Sum6/2
  Demux/1 -> Mux/1, Sum6/1
  Sum6/1 -> Mux/2
  ac/1 -> Demux/1

== system DPWMA_17_Level_Rectifier_Digital_PR/Subsystem/子模块1/Subsystem1 ==
  N : Inport
  MOD : Inport  Port=2
  AND : Logic  IconShape=distinctive  AllPortsSameDT=off  OutDataTypeStr=boolean
  AND1 : Logic  IconShape=distinctive  AllPortsSameDT=off  OutDataTypeStr=boolean
  OFFSET : Constant
  Relational Operator1 : RelationalOperator  Operator=<  OutDataTypeStr=boolean  InputSameDT=off
  Relational Operator2 : RelationalOperator  Operator=>  OutDataTypeStr=boolean  InputSameDT=off
  Relational Operator6 : RelationalOperator  Operator=>  OutDataTypeStr=boolean  InputSameDT=off
  Relational Operator7 : RelationalOperator  Operator=<  OutDataTypeStr=boolean  InputSameDT=off
  Sum1 : Sum  Inputs=|+-
  Sum2 : Sum  Inputs=|++
  Sum3 : Sum  Inputs=--|
  Sum4 : Sum  Inputs=++|
  Triangle1 : simulink/Sources/Repeating Sequence  rep_seq_t=[0 1/1800/2 1/1800]  rep_seq_y=[0 1 0]
  DRV1 : Outport
  DRV2 : Outport  Port=2
  wires:
  N/1 -> Sum3/1, Sum1/2
  MOD/1 -> Sum3/2, Sum1/1
  Sum1/1 -> Relational Operator7/1, Sum2/1
  Triangle1/1 -> Relational Operator2/2, Relational Operator1/2, Relational Operator6/2, Relational Operator7/2
  Sum2/1 -> Relational Operator6/1
  OFFSET/1 -> Sum2/2, Sum4/1
  Sum4/1 -> Relational Operator2/1
  Sum3/1 -> Relational Operator1/1, Sum4/2
  Relational Operator6/1 -> AND/2
  Relational Operator7/1 -> AND/1
  AND/1 -> DRV1/1
  Relational Operator1/1 -> AND1/1
  Relational Operator2/1 -> AND1/2
  AND1/1 -> DRV2/1

== system DPWMA_17_Level_Rectifier_Digital_PR/Subsystem/子模块2/Subsystem1 ==
  N : Inport
  MOD : Inport  Port=2
  AND : Logic  IconShape=distinctive  AllPortsSameDT=off  OutDataTypeStr=boolean
  AND1 : Logic  IconShape=distinctive  AllPortsSameDT=off  OutDataTypeStr=boolean
  OFFSET : Constant
  Relational Operator1 : RelationalOperator  Operator=<  OutDataTypeStr=boolean  InputSameDT=off
  Relational Operator2 : RelationalOperator  Operator=>  OutDataTypeStr=boolean  InputSameDT=off
  Relational Operator6 : RelationalOperator  Operator=>  OutDataTypeStr=boolean  InputSameDT=off
  Relational Operator7 : RelationalOperator  Operator=<  OutDataTypeStr=boolean  InputSameDT=off
  Sum1 : Sum  Inputs=|+-
  Sum2 : Sum  Inputs=|++
  Sum3 : Sum  Inputs=--|
  Sum4 : Sum  Inputs=++|
  Transport Delay : TransportDelay  DelayTime=1/3600/4
  Triangle1 : simulink/Sources/Repeating Sequence  rep_seq_t=[0 1/1800/2 1/1800]  rep_seq_y=[0 1 0]
  DRV1 : Outport
  DRV2 : Outport  Port=2
  wires:
  AND1/1 -> DRV2/1
  Relational Operator2/1 -> AND1/2
  Relational Operator1/1 -> AND1/1
  AND/1 -> DRV1/1
  Relational Operator7/1 -> AND/1
  Relational Operator6/1 -> AND/2
  Sum3/1 -> Sum4/2, Relational Operator1/1
  Sum4/1 -> Relational Operator2/1
  OFFSET/1 -> Sum4/1, Sum2/2
  Sum2/1 -> Relational Operator6/1
  Transport Delay/1 -> Relational Operator7/2, Relational Operator6/2, Relational Operator1/2, Relational Operator2/2
  Sum1/1 -> Sum2/1, Relational Operator7/1
  MOD/1 -> Sum1/1, Sum3/2
  N/1 -> Sum1/2, Sum3/1
  Triangle1/1 -> Transport Delay/1

== system DPWMA_17_Level_Rectifier_Digital_PR/Subsystem/子模块3/Subsystem1 ==
  N : Inport
  MOD : Inport  Port=2
  AND : Logic  IconShape=distinctive  AllPortsSameDT=off  OutDataTypeStr=boolean
  AND1 : Logic  IconShape=distinctive  AllPortsSameDT=off  OutDataTypeStr=boolean
  OFFSET : Constant
  Relational Operator1 : RelationalOperator  Operator=<  OutDataTypeStr=boolean  InputSameDT=off
  Relational Operator2 : RelationalOperator  Operator=>  OutDataTypeStr=boolean  InputSameDT=off
  Relational Operator6 : RelationalOperator  Operator=>  OutDataTypeStr=boolean  InputSameDT=off
  Relational Operator7 : RelationalOperator  Operator=<  OutDataTypeStr=boolean  InputSameDT=off
  Sum1 : Sum  Inputs=|+-
  Sum2 : Sum  Inputs=|++
  Sum3 : Sum  Inputs=--|
  Sum4 : Sum  Inputs=++|
  Transport Delay : TransportDelay  DelayTime=2/3600/4
  Triangle1 : simulink/Sources/Repeating Sequence  rep_seq_t=[0 1/1800/2 1/1800]  rep_seq_y=[0 1 0]
  DRV1 : Outport
  DRV2 : Outport  Port=2
  wires:
  Triangle1/1 -> Transport Delay/1
  N/1 -> Sum3/1, Sum1/2
  MOD/1 -> Sum3/2, Sum1/1
  Sum1/1 -> Relational Operator7/1, Sum2/1
  Transport Delay/1 -> Relational Operator2/2, Relational Operator1/2, Relational Operator6/2, Relational Operator7/2
  Sum2/1 -> Relational Operator6/1
  OFFSET/1 -> Sum2/2, Sum4/1
  Sum4/1 -> Relational Operator2/1
  Sum3/1 -> Relational Operator1/1, Sum4/2
  Relational Operator6/1 -> AND/2
  Relational Operator7/1 -> AND/1
  AND/1 -> DRV1/1
  Relational Operator1/1 -> AND1/1
  Relational Operator2/1 -> AND1/2
  AND1/1 -> DRV2/1

== system DPWMA_17_Level_Rectifier_Digital_PR/Subsystem/子模块4/Subsystem1 ==
  N : Inport
  MOD : Inport  Port=2
  AND : Logic  IconShape=distinctive  AllPortsSameDT=off  OutDataTypeStr=boolean
  AND1 : Logic  IconShape=distinctive  AllPortsSameDT=off  OutDataTypeStr=boolean
  OFFSET : Constant
  Relational Operator1 : RelationalOperator  Operator=<  OutDataTypeStr=boolean  InputSameDT=off
  Relational Operator2 : RelationalOperator  Operator=>  OutDataTypeStr=boolean  InputSameDT=off
  Relational Operator6 : RelationalOperator  Operator=>  OutDataTypeStr=boolean  InputSameDT=off
  Relational Operator7 : RelationalOperator  Operator=<  OutDataTypeStr=boolean  InputSameDT=off
  Sum1 : Sum  Inputs=|+-
  Sum2 : Sum  Inputs=|++
  Sum3 : Sum  Inputs=--|
  Sum4 : Sum  Inputs=++|
  Transport Delay : TransportDelay  DelayTime=3/3600/4
  Triangle1 : simulink/Sources/Repeating Sequence  rep_seq_t=[0 1/1800/2 1/1800]  rep_seq_y=[0 1 0]
  DRV1 : Outport
  DRV2 : Outport  Port=2
  wires:
  AND1/1 -> DRV2/1
  Relational Operator2/1 -> AND1/2
  Relational Operator1/1 -> AND1/1
  AND/1 -> DRV1/1
  Relational Operator7/1 -> AND/1
  Relational Operator6/1 -> AND/2
  Sum3/1 -> Sum4/2, Relational Operator1/1
  Sum4/1 -> Relational Operator2/1
  OFFSET/1 -> Sum4/1, Sum2/2
  Sum2/1 -> Relational Operator6/1
  Transport Delay/1 -> Relational Operator7/2, Relational Operator6/2, Relational Operator1/2, Relational Operator2/2
  Sum1/1 -> Sum2/1, Relational Operator7/1
  MOD/1 -> Sum1/1, Sum3/2
  N/1 -> Sum1/2, Sum3/1
  Triangle1/1 -> Transport Delay/1

== system DPWMA_17_Level_Rectifier_Digital_PR/Subsystem1/子模块1/Subsystem1 ==
  N : Inport
  MOD : Inport  Port=2
  AND : Logic  IconShape=distinctive  AllPortsSameDT=off  OutDataTypeStr=boolean
  AND1 : Logic  IconShape=distinctive  AllPortsSameDT=off  OutDataTypeStr=boolean
  OFFSET : Constant
  Relational Operator1 : RelationalOperator  Operator=<  OutDataTypeStr=boolean  InputSameDT=off
  Relational Operator2 : RelationalOperator  Operator=>  OutDataTypeStr=boolean  InputSameDT=off
  Relational Operator6 : RelationalOperator  Operator=>  OutDataTypeStr=boolean  InputSameDT=off
  Relational Operator7 : RelationalOperator  Operator=<  OutDataTypeStr=boolean  InputSameDT=off
  Sum1 : Sum  Inputs=|+-
  Sum2 : Sum  Inputs=|++
  Sum3 : Sum  Inputs=--|
  Sum4 : Sum  Inputs=++|
  Triangle1 : simulink/Sources/Repeating Sequence  rep_seq_t=[0 1/1800/2 1/1800]  rep_seq_y=[0 1 0]
  DRV1 : Outport
  DRV2 : Outport  Port=2
  wires:
  AND1/1 -> DRV2/1
  Relational Operator2/1 -> AND1/2
  Relational Operator1/1 -> AND1/1
  AND/1 -> DRV1/1
  Relational Operator7/1 -> AND/1
  Relational Operator6/1 -> AND/2
  Sum3/1 -> Sum4/2, Relational Operator1/1
  Sum4/1 -> Relational Operator2/1
  OFFSET/1 -> Sum4/1, Sum2/2
  Sum2/1 -> Relational Operator6/1
  Triangle1/1 -> Relational Operator7/2, Relational Operator6/2, Relational Operator1/2, Relational Operator2/2
  Sum1/1 -> Sum2/1, Relational Operator7/1
  MOD/1 -> Sum1/1, Sum3/2
  N/1 -> Sum1/2, Sum3/1

== system DPWMA_17_Level_Rectifier_Digital_PR/Subsystem1/子模块2/Subsystem1 ==
  N : Inport
  MOD : Inport  Port=2
  AND : Logic  IconShape=distinctive  AllPortsSameDT=off  OutDataTypeStr=boolean
  AND1 : Logic  IconShape=distinctive  AllPortsSameDT=off  OutDataTypeStr=boolean
  OFFSET : Constant
  Relational Operator1 : RelationalOperator  Operator=<  OutDataTypeStr=boolean  InputSameDT=off
  Relational Operator2 : RelationalOperator  Operator=>  OutDataTypeStr=boolean  InputSameDT=off
  Relational Operator6 : RelationalOperator  Operator=>  OutDataTypeStr=boolean  InputSameDT=off
  Relational Operator7 : RelationalOperator  Operator=<  OutDataTypeStr=boolean  InputSameDT=off
  Sum1 : Sum  Inputs=|+-
  Sum2 : Sum  Inputs=|++
  Sum3 : Sum  Inputs=--|
  Sum4 : Sum  Inputs=++|
  Transport Delay : TransportDelay  DelayTime=1/3600/4
  Triangle1 : simulink/Sources/Repeating Sequence  rep_seq_t=[0 1/1800/2 1/1800]  rep_seq_y=[0 1 0]
  DRV1 : Outport
  DRV2 : Outport  Port=2
  wires:
  Triangle1/1 -> Transport Delay/1
  N/1 -> Sum3/1, Sum1/2
  MOD/1 -> Sum3/2, Sum1/1
  Sum1/1 -> Relational Operator7/1, Sum2/1
  Transport Delay/1 -> Relational Operator2/2, Relational Operator1/2, Relational Operator6/2, Relational Operator7/2
  Sum2/1 -> Relational Operator6/1
  OFFSET/1 -> Sum2/2, Sum4/1
  Sum4/1 -> Relational Operator2/1
  Sum3/1 -> Relational Operator1/1, Sum4/2
  Relational Operator6/1 -> AND/2
  Relational Operator7/1 -> AND/1
  AND/1 -> DRV1/1
  Relational Operator1/1 -> AND1/1
  Relational Operator2/1 -> AND1/2
  AND1/1 -> DRV2/1

== system DPWMA_17_Level_Rectifier_Digital_PR/Subsystem1/子模块3/Subsystem1 ==
  N : Inport
  MOD : Inport  Port=2
  AND : Logic  IconShape=distinctive  AllPortsSameDT=off  OutDataTypeStr=boolean
  AND1 : Logic  IconShape=distinctive  AllPortsSameDT=off  OutDataTypeStr=boolean
  OFFSET : Constant
  Relational Operator1 : RelationalOperator  Operator=<  OutDataTypeStr=boolean  InputSameDT=off
  Relational Operator2 : RelationalOperator  Operator=>  OutDataTypeStr=boolean  InputSameDT=off
  Relational Operator6 : RelationalOperator  Operator=>  OutDataTypeStr=boolean  InputSameDT=off
  Relational Operator7 : RelationalOperator  Operator=<  OutDataTypeStr=boolean  InputSameDT=off
  Sum1 : Sum  Inputs=|+-
  Sum2 : Sum  Inputs=|++
  Sum3 : Sum  Inputs=--|
  Sum4 : Sum  Inputs=++|
  Transport Delay : TransportDelay  DelayTime=2/3600/4
  Triangle1 : simulink/Sources/Repeating Sequence  rep_seq_t=[0 1/1800/2 1/1800]  rep_seq_y=[0 1 0]
  DRV1 : Outport
  DRV2 : Outport  Port=2
  wires:
  AND1/1 -> DRV2/1
  Relational Operator2/1 -> AND1/2
  Relational Operator1/1 -> AND1/1
  AND/1 -> DRV1/1
  Relational Operator7/1 -> AND/1
  Relational Operator6/1 -> AND/2
  Sum3/1 -> Sum4/2, Relational Operator1/1
  Sum4/1 -> Relational Operator2/1
  OFFSET/1 -> Sum4/1, Sum2/2
  Sum2/1 -> Relational Operator6/1
  Transport Delay/1 -> Relational Operator7/2, Relational Operator6/2, Relational Operator1/2, Relational Operator2/2
  Sum1/1 -> Sum2/1, Relational Operator7/1
  MOD/1 -> Sum1/1, Sum3/2
  N/1 -> Sum1/2, Sum3/1
  Triangle1/1 -> Transport Delay/1

== system DPWMA_17_Level_Rectifier_Digital_PR/Subsystem1/子模块4/Subsystem1 ==
  N : Inport
  MOD : Inport  Port=2
  AND : Logic  IconShape=distinctive  AllPortsSameDT=off  OutDataTypeStr=boolean
  AND1 : Logic  IconShape=distinctive  AllPortsSameDT=off  OutDataTypeStr=boolean
  OFFSET : Constant
  Relational Operator1 : RelationalOperator  Operator=<  OutDataTypeStr=boolean  InputSameDT=off
  Relational Operator2 : RelationalOperator  Operator=>  OutDataTypeStr=boolean  InputSameDT=off
  Relational Operator6 : RelationalOperator  Operator=>  OutDataTypeStr=boolean  InputSameDT=off
  Relational Operator7 : RelationalOperator  Operator=<  OutDataTypeStr=boolean  InputSameDT=off
  Sum1 : Sum  Inputs=|+-
  Sum2 : Sum  Inputs=|++
  Sum3 : Sum  Inputs=--|
  Sum4 : Sum  Inputs=++|
  Transport Delay : TransportDelay  DelayTime=3/3600/4
  Triangle1 : simulink/Sources/Repeating Sequence  rep_seq_t=[0 1/1800/2 1/1800]  rep_seq_y=[0 1 0]
  DRV1 : Outport
  DRV2 : Outport  Port=2
  wires:
  Triangle1/1 -> Transport Delay/1
  N/1 -> Sum3/1, Sum1/2
  MOD/1 -> Sum3/2, Sum1/1
  Sum1/1 -> Relational Operator7/1, Sum2/1
  Transport Delay/1 -> Relational Operator2/2, Relational Operator1/2, Relational Operator6/2, Relational Operator7/2
  Sum2/1 -> Relational Operator6/1
  OFFSET/1 -> Sum2/2, Sum4/1
  Sum4/1 -> Relational Operator2/1
  Sum3/1 -> Relational Operator1/1, Sum4/2
  Relational Operator6/1 -> AND/2
  Relational Operator7/1 -> AND/1
  AND/1 -> DRV1/1
  Relational Operator1/1 -> AND1/1
  Relational Operator2/1 -> AND1/2
  AND1/1 -> DRV2/1

== system DPWMA_17_Level_Rectifier_Digital_PR/Subsystem2/子模块1/Subsystem1 ==
  N : Inport
  MOD : Inport  Port=2
  AND : Logic  IconShape=distinctive  AllPortsSameDT=off  OutDataTypeStr=boolean
  AND1 : Logic  IconShape=distinctive  AllPortsSameDT=off  OutDataTypeStr=boolean
  OFFSET : Constant
  Relational Operator1 : RelationalOperator  Operator=<  OutDataTypeStr=boolean  InputSameDT=off
  Relational Operator2 : RelationalOperator  Operator=>  OutDataTypeStr=boolean  InputSameDT=off
  Relational Operator6 : RelationalOperator  Operator=>  OutDataTypeStr=boolean  InputSameDT=off
  Relational Operator7 : RelationalOperator  Operator=<  OutDataTypeStr=boolean  InputSameDT=off
  Sum1 : Sum  Inputs=|+-
  Sum2 : Sum  Inputs=|++
  Sum3 : Sum  Inputs=--|
  Sum4 : Sum  Inputs=++|
  Triangle1 : simulink/Sources/Repeating Sequence  rep_seq_t=[0 1/1800/2 1/1800]  rep_seq_y=[0 1 0]
  DRV1 : Outport
  DRV2 : Outport  Port=2
  wires:
  N/1 -> Sum3/1, Sum1/2
  MOD/1 -> Sum3/2, Sum1/1
  Sum1/1 -> Relational Operator7/1, Sum2/1
  Triangle1/1 -> Relational Operator2/2, Relational Operator1/2, Relational Operator6/2, Relational Operator7/2
  Sum2/1 -> Relational Operator6/1
  OFFSET/1 -> Sum2/2, Sum4/1
  Sum4/1 -> Relational Operator2/1
  Sum3/1 -> Relational Operator1/1, Sum4/2
  Relational Operator6/1 -> AND/2
  Relational Operator7/1 -> AND/1
  AND/1 -> DRV1/1
  Relational Operator1/1 -> AND1/1
  Relational Operator2/1 -> AND1/2
  AND1/1 -> DRV2/1

== system DPWMA_17_Level_Rectifier_Digital_PR/Subsystem2/子模块2/Subsystem1 ==
  N : Inport
  MOD : Inport  Port=2
  AND : Logic  IconShape=distinctive  AllPortsSameDT=off  OutDataTypeStr=boolean
  AND1 : Logic  IconShape=distinctive  AllPortsSameDT=off  OutDataTypeStr=boolean
  OFFSET : Constant
  Relational Operator1 : RelationalOperator  Operator=<  OutDataTypeStr=boolean  InputSameDT=off
  Relational Operator2 : RelationalOperator  Operator=>  OutDataTypeStr=boolean  InputSameDT=off
  Relational Operator6 : RelationalOperator  Operator=>  OutDataTypeStr=boolean  InputSameDT=off
  Relational Operator7 : RelationalOperator  Operator=<  OutDataTypeStr=boolean  InputSameDT=off
  Sum1 : Sum  Inputs=|+-
  Sum2 : Sum  Inputs=|++
  Sum3 : Sum  Inputs=--|
  Sum4 : Sum  Inputs=++|
  Transport Delay : TransportDelay  DelayTime=1/3600/4
  Triangle1 : simulink/Sources/Repeating Sequence  rep_seq_t=[0 1/1800/2 1/1800]  rep_seq_y=[0 1 0]
  DRV1 : Outport
  DRV2 : Outport  Port=2
  wires:
  AND1/1 -> DRV2/1
  Relational Operator2/1 -> AND1/2
  Relational Operator1/1 -> AND1/1
  AND/1 -> DRV1/1
  Relational Operator7/1 -> AND/1
  Relational Operator6/1 -> AND/2
  Sum3/1 -> Sum4/2, Relational Operator1/1
  Sum4/1 -> Relational Operator2/1
  OFFSET/1 -> Sum4/1, Sum2/2
  Sum2/1 -> Relational Operator6/1
  Transport Delay/1 -> Relational Operator7/2, Relational Operator6/2, Relational Operator1/2, Relational Operator2/2
  Sum1/1 -> Sum2/1, Relational Operator7/1
  MOD/1 -> Sum1/1, Sum3/2
  N/1 -> Sum1/2, Sum3/1
  Triangle1/1 -> Transport Delay/1

== system DPWMA_17_Level_Rectifier_Digital_PR/Subsystem2/子模块3/Subsystem1 ==
  N : Inport
  MOD : Inport  Port=2
  AND : Logic  IconShape=distinctive  AllPortsSameDT=off  OutDataTypeStr=boolean
  AND1 : Logic  IconShape=distinctive  AllPortsSameDT=off  OutDataTypeStr=boolean
  OFFSET : Constant
  Relational Operator1 : RelationalOperator  Operator=<  OutDataTypeStr=boolean  InputSameDT=off
  Relational Operator2 : RelationalOperator  Operator=>  OutDataTypeStr=boolean  InputSameDT=off
  Relational Operator6 : RelationalOperator  Operator=>  OutDataTypeStr=boolean  InputSameDT=off
  Relational Operator7 : RelationalOperator  Operator=<  OutDataTypeStr=boolean  InputSameDT=off
  Sum1 : Sum  Inputs=|+-
  Sum2 : Sum  Inputs=|++
  Sum3 : Sum  Inputs=--|
  Sum4 : Sum  Inputs=++|
  Transport Delay : TransportDelay  DelayTime=2/3600/4
  Triangle1 : simulink/Sources/Repeating Sequence  rep_seq_t=[0 1/1800/2 1/1800]  rep_seq_y=[0 1 0]
  DRV1 : Outport
  DRV2 : Outport  Port=2
  wires:
  Triangle1/1 -> Transport Delay/1
  N/1 -> Sum3/1, Sum1/2
  MOD/1 -> Sum3/2, Sum1/1
  Sum1/1 -> Relational Operator7/1, Sum2/1
  Transport Delay/1 -> Relational Operator2/2, Relational Operator1/2, Relational Operator6/2, Relational Operator7/2
  Sum2/1 -> Relational Operator6/1
  OFFSET/1 -> Sum2/2, Sum4/1
  Sum4/1 -> Relational Operator2/1
  Sum3/1 -> Relational Operator1/1, Sum4/2
  Relational Operator6/1 -> AND/2
  Relational Operator7/1 -> AND/1
  AND/1 -> DRV1/1
  Relational Operator1/1 -> AND1/1
  Relational Operator2/1 -> AND1/2
  AND1/1 -> DRV2/1

== system DPWMA_17_Level_Rectifier_Digital_PR/Subsystem2/子模块4/Subsystem1 ==
  N : Inport
  MOD : Inport  Port=2
  AND : Logic  IconShape=distinctive  AllPortsSameDT=off  OutDataTypeStr=boolean
  AND1 : Logic  IconShape=distinctive  AllPortsSameDT=off  OutDataTypeStr=boolean
  OFFSET : Constant
  Relational Operator1 : RelationalOperator  Operator=<  OutDataTypeStr=boolean  InputSameDT=off
  Relational Operator2 : RelationalOperator  Operator=>  OutDataTypeStr=boolean  InputSameDT=off
  Relational Operator6 : RelationalOperator  Operator=>  OutDataTypeStr=boolean  InputSameDT=off
  Relational Operator7 : RelationalOperator  Operator=<  OutDataTypeStr=boolean  InputSameDT=off
  Sum1 : Sum  Inputs=|+-
  Sum2 : Sum  Inputs=|++
  Sum3 : Sum  Inputs=--|
  Sum4 : Sum  Inputs=++|
  Transport Delay : TransportDelay  DelayTime=3/3600/4
  Triangle1 : simulink/Sources/Repeating Sequence  rep_seq_t=[0 1/1800/2 1/1800]  rep_seq_y=[0 1 0]
  DRV1 : Outport
  DRV2 : Outport  Port=2
  wires:
  AND1/1 -> DRV2/1
  Relational Operator2/1 -> AND1/2
  Relational Operator1/1 -> AND1/1
  AND/1 -> DRV1/1
  Relational Operator7/1 -> AND/1
  Relational Operator6/1 -> AND/2
  Sum3/1 -> Sum4/2, Relational Operator1/1
  Sum4/1 -> Relational Operator2/1
  OFFSET/1 -> Sum4/1, Sum2/2
  Sum2/1 -> Relational Operator6/1
  Transport Delay/1 -> Relational Operator7/2, Relational Operator6/2, Relational Operator1/2, Relational Operator2/2
  Sum1/1 -> Sum2/1, Relational Operator7/1
  MOD/1 -> Sum1/1, Sum3/2
  N/1 -> Sum1/2, Sum3/1
  Triangle1/1 -> Transport Delay/1

== matlab function DPWMA_17_Level_Rectifier_Digital_PR/Digital PR A-C/Discrete PR ==
  settings: updateMethod=DISCRETE  sampleTime=Ts
  data: err_A input; err_C input; out_A output; Kp input; Kr input; Wc input; Ts input; out_C output
function [out_A, out_C] = fcn(err_A, err_C, Kp, Kr, Wc, Ts)

W0 = 50*2*pi;

%%定义三相静态变量
persistent err_A1;
persistent err_A2;
persistent out_A1;
persistent out_A2;

persistent err_C1;
persistent err_C2;
persistent out_C1;
persistent out_C2;

%%对三相静态变量初始化
if isempty(err_A1)
    err_A1 = 0;
end
if isempty(err_A2)
    err_A2 = 0;
end
if isempty(out_A1)
    out_A1 = 0;
end
if isempty(out_A2)
    out_A2 = 0;
end


if isempty(err_C1)
    err_C1 = 0;
end
if isempty(err_C2)
    err_C2 = 0;
end
if isempty(out_C1)
    out_C1 = 0;
end
if isempty(out_C2)
    out_C2 = 0;
end

%%Discrete
t1 = Wc * Ts;
t2 = W0^2 * Ts^2;
t3 = t2 + 4*t1 + 4;

b0 = (Kp*t2 + 4*(Kp+Kr)*t1 + 4*Kp) / t3;
b1 = (2*Kp*t2 - 8*Kp) / t3;
b2 = (Kp*t2 + 4*Kp - 4*(Kp+Kr)*t1) / t3;
a1 = (2*t2 - 8) / t3;
a2 = (t2 - 4*t1 + 4) / t3;
%%限制输出
if b0>3000
    b0=0;
end
if b0<-3000
    b0=0;
end

%%计算三相输出量
out_A = b0*err_A + b1*err_A1 + b2*err_A2 - a1*out_A1 - a2*out_A2;
out_A2 = out_A1;
out_A1 = out_A;
err_A2 = err_A1;
err_A1 = err_A;


out_C = b0*err_C + b1*err_C1 + b2*err_C2 - a1*out_C1 - a2*out_C2;
out_C2 = out_C1;
out_C1 = out_C;
err_C2 = err_C1;
err_C1 = err_C;
